simulink model "hdlcoder_int2bits_bits2int"  (R2026a)
settings: Solver=FixedStepDiscrete  StopTime=10
model workspace (MAT data in the model file):
  maxWordLength = 64
  u = embedded.fi
  u.DataType = 'Fixed'
  u.Scaling = 'BinaryPoint'
  u.Signed = 1
  u.WordLength = 16
  u.FixedExponent = -13
  u.SlopeAdjustmentFactor = 1
  u.Bias = 0
  u.DataTypeOverride = 'Inherit'
  u.intarray = -25736
  u.noverflows = 0
  u.nunderflows = 0
  u.maxlog = -1.79769313486e+308
  u.minlog = 1.79769313486e+308
  u.RoundingMethod = 'Nearest'
  u.OverflowAction = 'Saturate'
  u.ProductMode = 'FullPrecision'
  u.SumMode = 'FullPrecision'
  u.ProductWordLength = 32
  u.SumWordLength = 32
  u.MaxProductWordLength = 65535
  u.MaxSumWordLength = 65535
  u.ProductFractionLength = 30
  u.ProductFixedExponent = -30
  u.ProductSlope = 9.31322574615e-10
  u.ProductSlopeAdjustmentFactor = 1
  u.ProductBias = 0
  u.SumFractionLength = 30
  u.SumFixedExponent = -30
  u.SumSlope = 9.31322574615e-10
  u.SumSlopeAdjustmentFactor = 1
  u.SumBias = 0
  u.CastBeforeSum = 1
  u.DDGMaxProductWordLength = 65535
  u.DDGMaxSumWordLength = 65535
  u.DDGProductFixedExponent = -30
  u.DDGProductFractionLength = 30
  u.DDGProductWordLength = 32
  u.DDGSumFixedExponent = -30
  u.DDGSumFractionLength = 30
  u.DDGSumWordLength = 32
  u.DDGCastBeforeSum = 1
  u.DDGProductBias = 0
  u.DDGProductSlopeAdjustmentFactor = 1
  u.DDGSumBias = 0
  u.DDGSumSlopeAdjustmentFactor = 1
  u.DDGProductSlope = 9.31322574615e-10
  u.DDGSumSlope = 9.31322574615e-10
  u.Logging = 0
  u.fimathislocal = 0
settings Model: DataTypeOverride=Off  Creator=The MathWorks, Inc.  LastModifiedBy=The MathWorks, Inc.
settings OptimizationCC: ConditionallyExecuteInputs=off
settings DebuggingCC: AlgebraicLoopMsg=error  SingleTaskRateTransMsg=error  StrictBusMsg=ErrorOnBusTreatedAsVector
settings HardwareCC: ProdHWDeviceType=ASIC/FPGA->ASIC/FPGA  ProdEqTarget=off
settings ConfigComp: CovScope=ReferencedModels

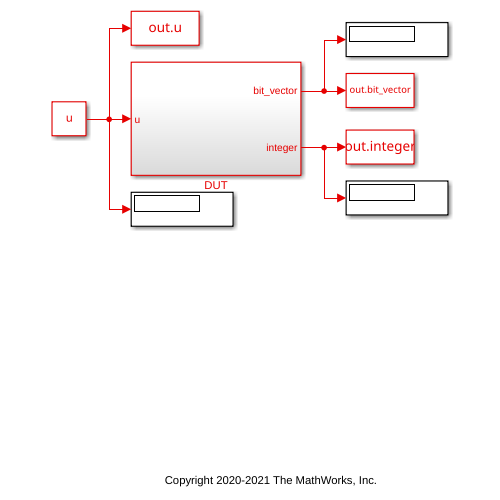
[thumbnail: Simulink's stored preview of the top-level diagram]
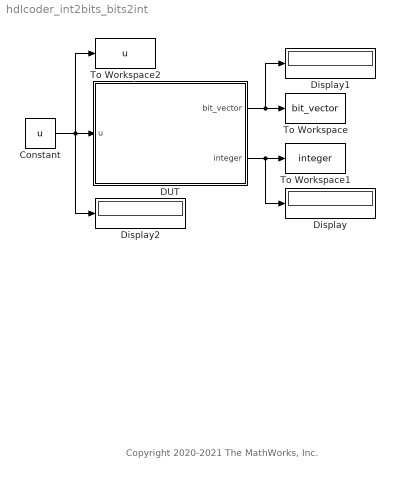
== system hdlcoder_int2bits_bits2int ==
  note: Copyright 2020-2021 The MathWorks, Inc.
  Constant : Constant  Value=u  SampleTime=1
  DUT : Subsystem
  Display : Display
  Display1 : Display
  Display2 : Display
  To Workspace : ToWorkspace  VariableName=bit_vector  SampleTime=1
      settings: MaxDataPoints=1
  To Workspace1 : ToWorkspace  VariableName=integer  SampleTime=1
      settings: MaxDataPoints=1
  To Workspace2 : ToWorkspace  VariableName=u  SampleTime=1
      settings: MaxDataPoints=1
  wires:
  DUT/1(bit_vector) -> To Workspace/1, Display1/1
  DUT/2(integer) -> To Workspace1/1, Display/1
  Constant/1 -> To Workspace2/1, Display2/1, DUT/1(u)

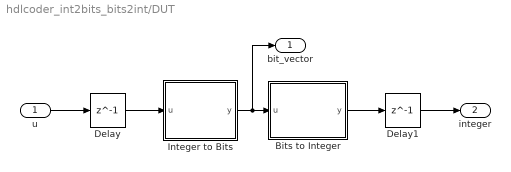
== system hdlcoder_int2bits_bits2int/DUT ==
  u : Inport
  Bits to Integer : MATLAB Function  TreatAsAtomicUnit=on
  Delay : Delay  DelayLength=1
  Delay1 : Delay  DelayLength=1
  Integer to Bits : Subsystem  mask{maxWordLength=maxWordLength}
      mask prompts: maxWordLength "Maximum Word Length"
      mask Display: disp('Integer to Bits')
  bit_vector : Outport
  integer : Outport  Port=2
  wires:
  Integer to Bits/1(y) -> Bits to Integer/1(u), bit_vector/1
  Delay/1 -> Integer to Bits/1(u)
  Bits to Integer/1(y) -> Delay1/1
  u/1 -> Delay/1
  Delay1/1 -> integer/1

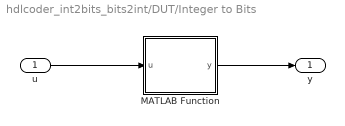
== system hdlcoder_int2bits_bits2int/DUT/Integer to Bits ==
  u : Inport
  MATLAB Function : MATLAB Function  TreatAsAtomicUnit=on
  y : Outport
  wires:
  u/1 -> MATLAB Function/1(u)
  MATLAB Function/1(y) -> y/1

== matlab function hdlcoder_int2bits_bits2int/DUT/Integer to Bits/MATLAB Function ==
  data: u input size=1; y output; maxWordLength parameter size=1
function y = integerToBits(u,maxWordLength)
    assert(isfi(u) && isfixed(u) && isscalar(u) && isreal(u));
    assert(u.WordLength <= maxWordLength)
    y = zeros(1,maxWordLength,'like',fi([],0,1,0));
    coder.unroll
    for k = 1:u.WordLength
        y(k) = bitsliceget(u, k, k);
    end
end

== matlab function hdlcoder_int2bits_bits2int/DUT/Bits to Integer ==
  data: u input; y output
function y = bitsToInteger(u)
    assert(isfi(u) && isfixed(u) && isvector(u) && isreal(u));
    w = length(u);
    y = fi(0,0,w,0);
    coder.unroll
    for k = 1:w
        y = bitset(y, k, u(k));
    end
end
